simulink library "rangefinders_lib"  (R2018b)
settings: Solver=VariableStepAuto  StartTime=0.0  StopTime=10.0  RelTol=1e-3
libraries: vrlib x1
settings Model: Creator=fabian  LastModifiedBy=yannic

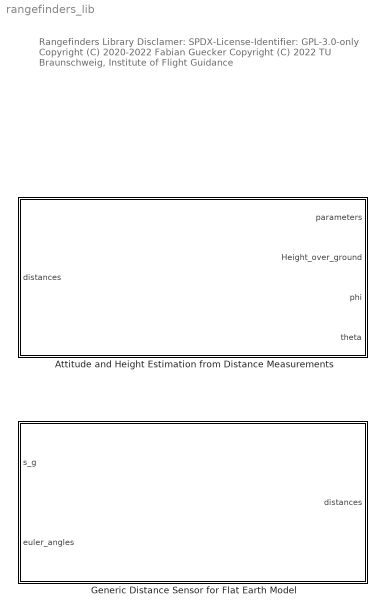
== system rangefinders_lib ==
  note: Rangefinders Library
      |
      | Disclamer:
      | SPDX-License-Identifier: GPL-3.0-only
      |
      | Copyright (C) 2020-2022 Fabian Guecker
      | Copyright (C) 2022 TU Braunschweig, Institute of Flight Guidance
  Attitude and Height Estimation from Distance Measurements : Subsystem  mask{theta=[-75 -75 -75], psi=[0 90 -90]}
      mask prompts: theta "Nickwinkel"; psi "Gierwinkel"
      mask init:
      | size_n = length(theta);
      | 
      | A = zeros(size_n,3)
      | 
      | for i = 1:size_n
      |     A(i,:) = (euler2Dcm(pi/180*[0 theta(i) psi(i)])' * [1; 0; 0])';
      | end
      | 
      | A_inv = inv(A);
      | 
      | d = ones(size_n, 1)
  Generic Distance Sensor for Flat Earth Model : Subsystem  mask{theta=[-75 -75 -75], psi=[0 90 -90], range=[60 60 60]}
      mask prompts: theta "Nickwinkel"; psi "Gierwinkel"

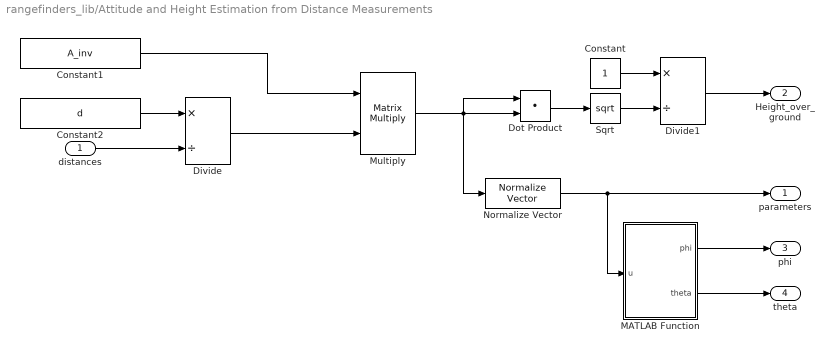
== system rangefinders_lib/Attitude and Height Estimation from Distance Measurements ==
  distances : Inport
  Constant : Constant
  Constant1 : Constant  Value=A_inv  VectorParams1D=off
  Constant2 : Constant  Value=d  VectorParams1D=off
  Divide : Product  Inputs=*/
  Divide1 : Product  Inputs=*/
  Dot Product : DotProduct  InputSameDT=on  OutDataTypeStr=Inherit: Inherit via internal rule
  MATLAB Function : MATLAB Function  TreatAsAtomicUnit=on
  Multiply : Product  Multiplication=Matrix(*)
  Normalize Vector : vrlib/Utilities/Normalize Vector  maxzero=0
      settings: SourceProductName=Simulink 3D Animation  SourceProductBaseCode=VR
  Sqrt : Sqrt  SaturateOnIntegerOverflow=on
  parameters : Outport
  Height_over_ground : Outport  Port=2
  phi : Outport  Port=3
  theta : Outport  Port=4
  wires:
  Constant1/1 -> Multiply/1
  Constant2/1 -> Divide/1
  distances/1 -> Divide/2
  Divide/1 -> Multiply/2
  Multiply/1 -> Dot Product/1, Normalize Vector/1, Dot Product/2
  Dot Product/1 -> Sqrt/1
  Sqrt/1 -> Divide1/2
  Divide1/1 -> Height_over_ground/1
  Constant/1 -> Divide1/1
  Normalize Vector/1 -> MATLAB Function/1(u), parameters/1
  MATLAB Function/1(phi) -> phi/1
  MATLAB Function/2(theta) -> theta/1

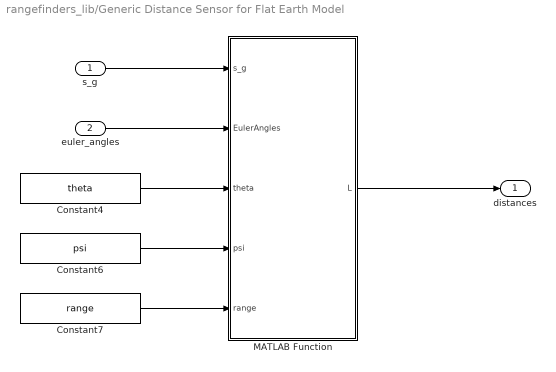
== system rangefinders_lib/Generic Distance Sensor for Flat Earth Model ==
  s_g : Inport
  euler_angles : Inport  Port=2
  Constant4 : Constant  Value=theta  VectorParams1D=off
  Constant6 : Constant  Value=psi  VectorParams1D=off
  Constant7 : Constant  Value=range  VectorParams1D=off
  MATLAB Function : MATLAB Function  TreatAsAtomicUnit=on
  distances : Outport
  wires:
  MATLAB Function/1(L) -> distances/1
  Constant7/1 -> MATLAB Function/5(range)
  s_g/1 -> MATLAB Function/1(s_g)
  euler_angles/1 -> MATLAB Function/2(EulerAngles)
  Constant4/1 -> MATLAB Function/3(theta)
  Constant6/1 -> MATLAB Function/4(psi)

== matlab function rangefinders_lib/Attitude and Height Estimation from Distance Measurements/MATLAB Function ==
  data: u input; phi output; theta output
function [phi,theta] = fcn(u)

phi   = atan2(u(2), u(3));
theta = atan2(-u(1), sqrt(u(2)^2 + u(3)^2));

end

== matlab function rangefinders_lib/Generic Distance Sensor for Flat Earth Model/MATLAB Function ==
  data: s_g input; EulerAngles input; theta input; psi input; L output; range input
function L  = calc_length(s_g,EulerAngles,theta,psi,range)

n  = [0 0 1];
V0 = [0 0 0];
P0 = [0 0 s_g(3)];

M_bg = euler2Dcm(EulerAngles);

L = zeros(length(theta),1);

for i=1:length(theta)
    matrix_rot_T  = euler2Dcm(pi/180*[0 theta(i) psi(i)])';
    normal_vector = matrix_rot_T * [range(i); 0; 0];
    u = (M_bg' * normal_vector)';
    L(i) = plane_line_intersect(n,V0,P0,u);
end


end

function L = plane_line_intersect(n,V0,P0,u)

L = 60;
I = [0 0 0];
P1 = P0 + u ;
w = P0 - V0;
D = dot(n,u);
N = -dot(n,w);
if abs(D) < 10^-7
    return;
end

sI = N / D;
I = P0 + sI.*u;
if (sI < 0 || sI > 1)
    L = norm(P0-P1);
else
    L = norm(I-P0);
end

end
